simulink model "VTS_challenge_2021"  (R2019b)
settings: Solver=ode1  StartTime=0.0  StopTime=SIMULPARAM.T_end  FixedStep=SIMULPARAM.Ts  RelTol=1e-3
undefined symbols (not defined in the file or in its folder): BAT, CHAp, EM1, EM2, EMS, MTp, RDp, Speed_control, SPEEDCONTROL
libraries: simulink x3
(part 2 of 2)

== matlab function VTS_challenge_2021/EMS/MATLAB Function ==
  settings: updateMethod=DISCRETE
  data: F_trac_ref input; k_fr output; T_EDf_trac_max input; T_EDr_trac_max input; vehicle_speed input; T_f_regen_max input; T_r_regen_max input
function k_fr = PSO_kfr(F_trac_ref, T_EDf_trac_max, T_EDr_trac_max, vehicle_speed, T_f_regen_max, T_r_regen_max)
%#codegen
% ANLPSO-based EMS for IEEE VTS 2021 - Dual gear ratios: front 3.0, rear 4.0
% Based on Scolaro et al. 2021, with improvements for separate gear ratios

%% ===== VEHICLE / DRIVETRAIN PARAMETERS =====
R_w = 0.38;          % Wheel radius [m]
i_g_f = 3.0;         % Gear ratio FRONT axle
i_g_r = 4.0;         % Gear ratio REAR axle
eta_t = 0.95;        % Transmission efficiency (constant)

%% ===== ANLPSO PARAMETERS (improved from Table I) =====
N_PART = 100;        % Increased for better exploration
MAX_IT = 20;         % Increased slightly for accuracy
XI_MAX = 0.9;
XI_MIN = 0.3;
C1_MIN = 1.2;
C1_MAX = 1.8;
C = 3;

%% ===== PENALTY =====
GAMMA = 8000;        % Increased to enforce torque constraints strictly

%% ===== FORCE LIMITS (separate for front/rear) =====
F_f_max = (T_EDf_trac_max * i_g_f * eta_t) / R_w;
F_r_max = (T_EDr_trac_max * i_g_r * eta_t) / R_w;
F_req_abs = abs(F_trac_ref);

%% ===== DYNAMIC k_fr BOUNDS (improved Eq. 4-6) =====
margin_f = 0.98;     % Front margin
margin_r = 0.94;     % Tighter for rear (to prevent violation)

if F_req_abs < 1e-3
    k_min = 0.0;
    k_max = 1.0;
else
    if F_trac_ref >= 0  % Traction
        F_trac_ref_max = min(F_req_abs, F_f_max + F_r_max);
        k_min = max(0.0, 1.0 - (F_r_max * margin_r) / F_trac_ref_max);
        k_max = min(1.0, (F_f_max * margin_f) / F_trac_ref_max);
    else  % Braking/Regen - use reduced torque limits
        F_f_regen_max = (T_f_regen_max * i_g_f * eta_t) / R_w;
        F_r_regen_max = (T_r_regen_max * i_g_r * eta_t) / R_w;
        F_brake_max = F_f_regen_max + F_r_regen_max;
        F_req_brake = min(F_req_abs, F_brake_max);
        k_min = max(0.0, 1.0 - (F_r_regen_max * margin_r) / F_req_brake);
        k_max = min(1.0, (F_f_regen_max * margin_f) / F_req_brake);
    end
end
if k_min > k_max
    k_min = 0.0; k_max = 1.0;
end

%% ===== INITIALIZATION (Eq. 10-11) =====
kfr = zeros(N_PART, 1);
for i = 1:N_PART
    kfr(i) = k_min + (i-1)*(k_max - k_min)/(N_PART) + rand()*(k_max - k_min)/N_PART;
end
v = (k_max - k_min)/4 * (2*rand(N_PART,1) - 1);

pbest = kfr;
pbest_fit = -Inf * ones(N_PART,1);  % Maximize eta  
gbest = kfr(1);
gbest_fit = -Inf;

%% ===== INITIAL FITNESS =====
for i = 1:N_PART
    [T_f_req, T_r_req] = computeTorques(kfr(i), F_trac_ref, R_w, i_g_f, i_g_r, eta_t);
    omega_f = (vehicle_speed / R_w) * i_g_f;  % Motor angular speed front [rad/s]
    omega_r = (vehicle_speed / R_w) * i_g_r;  % Rear
    eta_f = getEfficiencyFront(T_f_req, omega_f);
    eta_r = getEfficiencyRear(T_r_req, omega_r);
    pbest_fit(i) = fitness(eta_f, eta_r, kfr(i), T_f_req, T_r_req, T_EDf_trac_max, T_EDr_trac_max, GAMMA);
    if pbest_fit(i) > gbest_fit
        gbest_fit = pbest_fit(i);
        gbest = kfr(i);
    end
end

%% ===== MAIN LOOP =====
for it = 1:MAX_IT
    xi = XI_MAX - ((it-1)/(MAX_IT-1))^0.5 * (XI_MAX - XI_MIN);
    
    eta_avg = mean(pbest_fit);
    eta_min = min(pbest_fit);
    c1 = zeros(N_PART,1); c2 = zeros(N_PART,1);
    for i = 1:N_PART
        if pbest_fit(i) < eta_avg
            c1(i) = C1_MAX - (C1_MAX - C1_MIN) * (pbest_fit(i) - eta_min) / (eta_avg - eta_min + eps);
        else
            c1(i) = C1_MIN;
        end
        c2(i) = C - c1(i);
    end
    
    for i = 1:N_PART
        r1 = rand(); r2 = rand();
        v(i) = xi * v(i) + c1(i)*r1*(pbest(i) - kfr(i)) + c2(i)*r2*(gbest - kfr(i));
        
        % Velocity clamping (improvement for stability)
        v_max = 0.2 * (k_max - k_min);
        v(i) = max(min(v(i), v_max), -v_max);
        
        kfr(i) = kfr(i) + v(i);
        kfr(i) = max(min(kfr(i), k_max), k_min);
        
        [T_f_req, T_r_req] = computeTorques(kfr(i), F_trac_ref, R_w, i_g_f, i_g_r, eta_t);
        omega_f = (vehicle_speed / R_w) * i_g_f;
        omega_r = (vehicle_speed / R_w) * i_g_r;
        eta_f = getEfficiencyFront(T_f_req, omega_f);
        eta_r = getEfficiencyRear(T_r_req, omega_r);
        fit = fitness(eta_f, eta_r, kfr(i), T_f_req, T_r_req, T_EDf_trac_max, T_EDr_trac_max, GAMMA);
        
        if fit > pbest_fit(i)
            pbest_fit(i) = fit;
            pbest(i) = kfr(i);
        end
        if fit > gbest_fit
            gbest_fit = fit;
            gbest = kfr(i);
        end
    end
    
    % Early stopping improved
    if max(pbest_fit) - min(pbest_fit) < 1e-5 || (it > 10 && std(pbest_fit) < 1e-6)
        break;
    end
end

k_fr = min(max(gbest, k_min), k_max);

end

%% ===== FITNESS (with stronger rear penalty) =====
function J = fitness(eta_f, eta_r, k_fr, T_f_req, T_r_req, T_f_max, T_r_max, GAMMA)
    if eta_f <= 0 || eta_r <= 0
        eta_total = 0;
    else
        eta_total = 1 / (k_fr / eta_f + (1 - k_fr) / eta_r);
    end
    penalty = 0;
    if abs(T_f_req) > T_f_max
        penalty = penalty + GAMMA * (abs(T_f_req) - T_f_max)^2;
    end
    if abs(T_r_req) > T_r_max
        penalty = penalty + 1.5 * GAMMA * (abs(T_r_req) - T_r_max)^2;  % Heavier on rear
    end
    J = eta_total - penalty;
end

%% ===== TORQUES COMPUTATION =====
function [T_f_req, T_r_req] = computeTorques(k_fr, F_trac_ref, R_w, i_g_f, i_g_r, eta_t)
    F_f = k_fr * F_trac_ref;
    F_r = (1 - k_fr) * F_trac_ref;
    T_f_req = (F_f * R_w) / (i_g_f * eta_t);
    T_r_req = (F_r * R_w) / (i_g_r * eta_t);
end

%% ===== EFFICIENCY PLACEHOLDERS =====
function eta = getEfficiencyFront(torque, omega)
    eta = 0.95;
end

function eta = getEfficiencyRear(torque, omega)
    eta = 0.95;
end
